simulink model "bms_vcu_inverter_can_simulink"  (R2025b)
settings: Solver=VariableStepAuto  StartTime=0.0  StopTime=6000  RelTol=1e-3
undefined symbols (not defined in the file): Ireq, Qcell, R0cell, R1cell, R2cell, SOC0, tau1, tau2
libraries: nesl_utility x6, canmsglib x6, simulink x4, fl_lib x4, batteryecm_lib x1
settings Model: Creator=User  LastModifiedBy=User

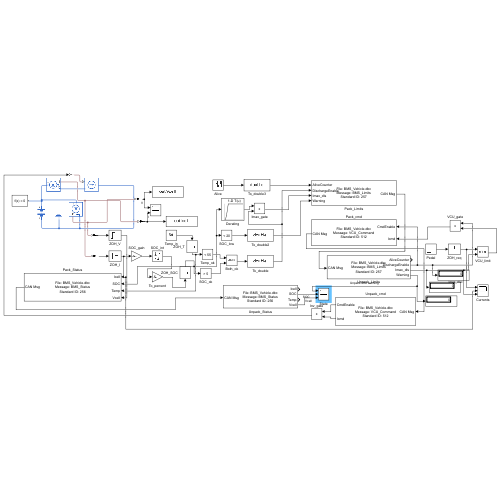
[thumbnail: Simulink's stored preview of the top-level diagram]
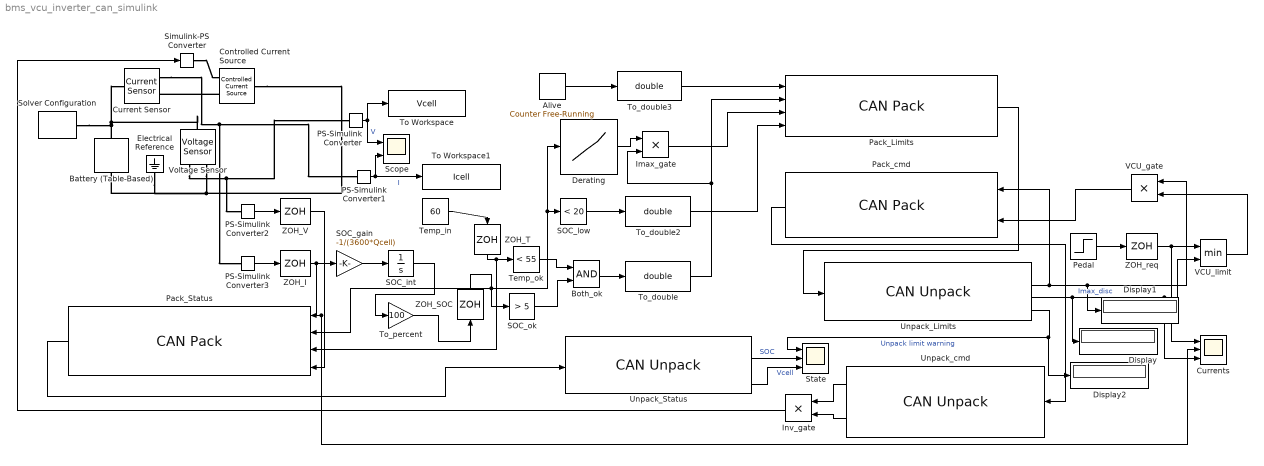
== system bms_vcu_inverter_can_simulink ==
  Alive : simulink/Sources/Counter Free-Running  NumBits=8  tsamp=0.1
  Battery (Table-Based) : batteryecm_lib/Battery (Table-Based)  SOC_vec=[0 0.2 0.5 0.8 1.0]  T_dependence=simscape.enum.tablebattery.temperature_dependence.no  prm_dir=simscape.enum.tablebattery.prm_dir.noCurrentDirectionality  T_vec=[278, 293, 313] K  V0_mat=[3.49, 3.5, 3.51; 3.55, 3.57, 3.56; 3.62, 3.63, 3.64; 3.71, 3.71, 3.72; 3.91, 3.93, 3.94; 4.07, 4.08, 4.08; 4.19, 4.19, 4.19] V  V0_vec=[3.0 3.5 3.7 4.0 4.2] V  V_range=[0, inf] V  R0_mat=[.0117, .0085, .009; .011, .0085, .009; .0114, .0087, .0092; .0107, .0082, .0088; .0107, .0083, .0091; .0113, .0085, .0089; .0116, .0085, .0089] Ohm  R0_vec=R0cell*ones(1,5) Ohm  R0_dis_mat=[.0117, .0085, .009; .011, .0085, .009; .0114, .0087, .0092; .0107, .0082, .0088; .0107, .0083, .0091; .0113, .0085, .0089; .0116, .0085, .0089] Ohm  R0_dis_vec=[.0085, .0085, .0087, .0082, .0083, .0085, .0085] Ohm  R0_ch_mat=[.0117, .0085, .009; .011, .0085, .009; .0114, .0087, .0092; .0107, .0082, .0088; .0107, .0083, .0091; .0113, .0085, .0089; .0116, .0085, .0089] Ohm  R0_ch_vec=[.0085, .0085, .0087, .0082, .0083, .0085, .0085] Ohm  AH=Qcell A*hr  prm_leak=simscape.enum.tablebattery.prm_leak.disabled  Rleak_vec=[8000, 7000, 6000] Ohm  Rleak=7e3 Ohm  extrapolation_option=simscape.enum.extrapolation.nearest  SOC_port=simscape.enum.tablebattery.enable.no  prm_dyn=simscape.enum.tablebattery.prm_dyn.rc2  R1_mat=[.0109, .0029, .0013; .0069, .0024, .0012; .0047, .0026, .0013; .0034, .0016, .001; .0033, .0023, .0014; .0033, .0018, .0011; .0028, .0017, .0011] Ohm  R1_vec=R1cell*ones(1,5) Ohm  tau1_mat=[20, 36, 39; 31, 45, 39; 109, 105, 61; 36, 29, 26; 59, 77, 67; 40, 33, 29; 25, 39, 33] s  tau1_vec=tau1*ones(1,5) s  R2_mat=[.0109, .0029, .0013; .0069, .0024, .0012; .0047, .0026, .0013; .0034, .0016, .001; .0033, .0023, .0014; .0033, .0018, .0011; .0028, .0017, .0011] Ohm  R2_vec=R2cell*ones(1,5) Ohm  tau2_mat=[20, 36, 39; 31, 45, 39; 109, 105, 61; 36, 29, 26; 59, 77, 67; 40, 33, 29; 25, 39, 33] s  tau2_vec=tau2*ones(1,5) s  R3_mat=[.0109, .0029, .0013; .0069, .0024, .0012; .0047, .0026, .0013; .0034, .0016, .001; .0033, .0023, .0014; .0033, .0018, .0011; .0028, .0017, .0011] Ohm  R3_vec=[.0029, .0024, .0026, .0016, .0023, .0018, .0017] Ohm  tau3_mat=[20, 36, 39; 31, 45, 39; 109, 105, 61; 36, 29, 26; 59, 77, 67; 40, 33, 29; 25, 39, 33] s  tau3_vec=[36, 45, 105, 29, 77, 33, 39] s  R4_mat=[.0109, .0029, .0013; .0069, .0024, .0012; .0047, .0026, .0013; .0034, .0016, .001; .0033, .0023, .0014; .0033, .0018, .0011; .0028, .0017, .0011] Ohm  R4_vec=[.0029, .0024, .0026, .0016, .0023, .0018, .0017] Ohm  tau4_mat=[20, 36, 39; 31, 45, 39; 109, 105, 61; 36, 29, 26; 59, 77, 67; 40, 33, 29; 25, 39, 33] s  tau4_vec=[36, 45, 105, 29, 77, 33, 39] s  R5_mat=[.0109, .0029, .0013; .0069, .0024, .0012; .0047, .0026, .0013; .0034, .0016, .001; .0033, .0023, .0014; .0033, .0018, .0011; .0028, .0017, .0011] Ohm  R5_vec=[.0029, .0024, .0026, .0016, .0023, .0018, .0017] Ohm  tau5_mat=[20, 36, 39; 31, 45, 39; 109, 105, 61; 36, 29, 26; 59, 77, 67; 40, 33, 29; 25, 39, 33] s  tau5_vec=[36, 45, 105, 29, 77, 33, 39] s  prm_fade=simscape.enum.tablebattery.prm_fade.disabled  N0=100  dV0=0  dR0=0  dAH=0  dRleak=0  dR1=0  dR2=0  dR3=0  dR4=0  dR5=0  N0vec=[0, 100, 200, 300]  Tfadevec=[298.15, 323.15] K  dV0vec=[0, 0, 0, 0]  dR0vec=[0, 0, 0, 0]  dAHvec=[0, 0, 0, 0]  dRleakvec=[0, 0, 0, 0]  dR1vec=[0, 0, 0, 0]  dR2vec=[0, 0, 0, 0]  dR3vec=[0, 0, 0, 0]  dR4vec=[0, 0, 0, 0]  dR5vec=[0, 0, 0, 0]  dV0mat=[0, 0; 0, 0; 0, 0; 0, 0]  dR0mat=[0, 0; 0, 0; 0, 0; 0, 0]  dAHmat=[0, 0; 0, 0; 0, 0; 0, 0]  dRleakmat=[0, 0; 0, 0; 0, 0; 0, 0]  dR1mat=[0, 0; 0, 0; 0, 0; 0, 0]  dR2mat=[0, 0; 0, 0; 0, 0; 0, 0]  dR3mat=[0, 0; 0, 0; 0, 0; 0, 0]  dR4mat=[0, 0; 0, 0; 0, 0; 0, 0]  dR5mat=[0, 0; 0, 0; 0, 0; 0, 0]  prm_age_modeling=simscape.enum.tablebattery.prm_age_modeling.equation  storage_dt_age_vec=[0] d  storage_T_age_vec=[273] K  prm_age_OCV=simscape.enum.tablebattery.prm_age_OCV.OCV  OCV_age=0.9  SOC_age=0.6  prm_age_resistance=simscape.enum.tablebattery.prm_age.disabled  OCV_scaling_age_resistance=2.2134e6  OCV_offset_age_resistance=1.632e6  temp_exp_age_resistance=0.515833569 V  t_exp_age_resistance=0.75  T_age_vec_resistance=[273.15, 298.15, 323.15] K  dt_age_vec_resistance=[0, 90, 180, 270] d  dR0_age_vec=[0, 0, 0]  t_meas_dR0_age=100 d  dR0_age_mat=[0, 0, 0; 0, 0, 0; 0, 0, 0; 0, 0, 0]  prm_age_capacity=simscape.enum.tablebattery.prm_age.disabled  OCV_scaling_age_capacity=1.5097e07  OCV_offset_age_capacity=8.3625e06  temp_exp_age_capacity=0.6011 V  t_exp_age_capacity=0.75  T_age_vec_capacity=[273.15, 298.15, 323.15] K  dt_age_vec_capacity=[0, 90, 180, 270] d  dAH_age_vec=[0, 0, 0]  t_meas_dAH_age=100 d  dAH_age_mat=[0, 0, 0; 0, 0, 0; 0, 0, 0; 0, 0, 0]  thermal_port=simscape.enum.thermaleffects.omit  temperature=298.15 K  thermal_mass=100 J/K  i_specify=off  i_priority=None  i=0 A  i_nominal_specify=off  i_nominal_value=1  i_nominal_unit=A  v_specify=off  v_priority=None  v=0 V  v_nominal_specify=off  v_nominal_value=1  v_nominal_unit=V  stateOfCharge_specify=on  stateOfCharge_priority=High  stateOfCharge=SOC0  stateOfCharge_nominal_specify=off  stateOfCharge_nominal_value=1  stateOfCharge_nominal_unit=1  num_cycles_specify=off  num_cycles_priority=High  num_cycles=0  num_cycles_nominal_specify=off  num_cycles_nominal_value=1  num_cycles_nominal_unit=1  cell_temperature_specify=off  cell_temperature_priority=High  cell_temperature=298.15 K  cell_temperature_nominal_specify=off  cell_temperature_nominal_value=1  cell_temperature_nominal_unit=K
      settings: InternalSimscapePortConfiguration="{\"Bottom\":[],\"Left\":[{\"id\":\"p\",\"label\":\"+\",\"type\":\"foundation.electrical.electrical\"}],\"Right\":[{\"id\":\"n\",\"label\":\"-\",\"type\":\"foundation.electrical.electrical\"}],\"Top\":[]}"
      settings: LibrarySourceBlock=|
      | batt_lib/Cells/Battery
      | (Table-Based)
  Both_ok : Logic  AllPortsSameDT=off  OutDataTypeStr=boolean
  Controlled Current Source : fl_lib/Electrical/Electrical Sources/Controlled Current Source
  Current Sensor : fl_lib/Electrical/Electrical Sensors/Current Sensor
  Currents : Scope  NumInputPorts=3
      settings: ActiveDisplayYMinimum=-0.74999999999999978  ActiveDisplayYMaximum=6.75
  Derating : Lookup_n-D  NumberOfTableDimensions=1  BreakpointsForDimension1=[0 5 10 20 100]  Table=[0 0 1.5 6 6]  InternalRulePriority=Speed  RndMeth=Simplest
  Display : Display
  Display1 : Display
  Display2 : Display
  Electrical Reference : fl_lib/Electrical/Electrical Elements/Electrical Reference
  Imax_gate : Product
  Inv_gate : Product
  PS-Simulink Converter{,1..3} (4 alike) : nesl_utility/PS-Simulink Converter  PhysicalDomain=network_engine_domain  SubClassName=ps_output  LeftPortType=input  RightPortType=output  PseudoPeriodic=off  Frequencies=[]  VectorFormat=inherit  Unit=inherit  AffineConversion=off
  Pack_Limits : canmsglib/CAN Pack  CANdbFile=C:\Users\User\Documents\MATLAB\BMS_Vehicle.dbc  MsgList=BMS_Limits  MsgName=BMS_Limits  MsgIDType=Standard (11-bit identifier)  MsgIdentifier=257  CANIDInput=off  MsgLength=8  Remote=off  ApplyMinMax=off  BusOutput=off  SignalInfo={'AliveCounter','32','8','LE','unsigned','Standard','0','1','0','0','255';'DischargeEnable','16','8','LE','unsigned','Standard','0','1','0','0','1';'Imax_dis','0','16','LE','unsigned','Standard','0','0.1','0','0','6553.5';'Warning','24','8','LE','unsigned','Standard','0','1','0','0','3'}
      settings: LibrarySourceBlock=c2000lib/Target Communication/CAN Pack  DataFormat=CANdb specified signals
  Pack_Status : canmsglib/CAN Pack  CANdbFile=C:\Users\User\Documents\MATLAB\BMS_Vehicle.dbc  MsgList=BMS_Status  MsgName=BMS_Status  MsgIDType=Standard (11-bit identifier)  MsgIdentifier=256  CANIDInput=off  MsgLength=8  Remote=off  ApplyMinMax=off  BusOutput=off  SignalInfo={'Icell','16','16','LE','signed','Standard','0','0.1','0','-3276.8','3276.7';'SOC','32','8','LE','unsigned','Standard','0','0.5','0','0','127.5';'Temp','40','8','LE','unsigned','Standard','0','1','-40','-40','215';'Vcell','0','16','LE','unsigned','Standard','0','0.001','0','0','65.535'}
      settings: LibrarySourceBlock=c2000lib/Target Communication/CAN Pack  DataFormat=CANdb specified signals
  Pack_cmd : canmsglib/CAN Pack  CANdbFile=C:\Users\User\Documents\MATLAB\BMS_Vehicle.dbc  MsgList=VCU_Command  MsgName=VCU_Command  MsgIDType=Standard (11-bit identifier)  MsgIdentifier=512  CANIDInput=off  MsgLength=8  Remote=off  ApplyMinMax=off  BusOutput=off  SignalInfo={'CmdEnable','16','8','LE','unsigned','Standard','0','1','0','0','1';'Icmd','0','16','LE','unsigned','Standard','0','0.1','0','0','6553.5'}
      settings: LibrarySourceBlock=c2000lib/Target Communication/CAN Pack  DataFormat=CANdb specified signals
  Pedal : Step  Time=10  After=Ireq  SampleTime=0
  SOC_gain : Gain  Gain=-1/(3600*Qcell)
  SOC_int : Integrator  InitialCondition=SOC0  LimitOutput=on  UpperSaturationLimit=1  LowerSaturationLimit=0
  SOC_low : simulink/Logic and Bit Operations/Compare To Constant  relop=<  const=20  OutDataTypeStr=boolean
  SOC_ok : simulink/Logic and Bit Operations/Compare To Constant  relop=>  const=5  OutDataTypeStr=boolean
  Scope : Scope  NumInputPorts=2
      settings: ActiveDisplayYMinimum=3.598991707315359  ActiveDisplayYMaximum=4.2008919512210277
  Simulink-PS Converter : nesl_utility/Simulink-PS Converter  PhysicalDomain=network_engine_domain  SubClassName=ps_input  LeftPortType=input  RightPortType=output  PseudoPeriodic=off  Frequencies=[]  NoiseDistribution=none  NoiseParameters=[]  Unit=1  AffineConversion=off  FilteringAndDerivatives=provide  SimscapeFilterOrder=1  InputFilterTimeConstant=0.001  UdotUserProvided=0
  Solver Configuration : nesl_utility/Solver Configuration  PhysicalDomain=network_engine_domain  SubClassName=solver  LeftPortType=input  RightPortType=generic  Tones=[]  Harmonics=[]  SimulateNoise=off  Profile=off  UseLocalSampling=off  EnableSwitchedLinearOptims=on  FrequencyDomain=off  UseCCode=off  RelTol=0.001  AbsTol=0.001  MinStep=1e-09  ToWorkspace=off  RevertToSquareIcSolve=off  NumHomotopyIterations=100  PhasorMode=off  PhasorModeNumHarmonics=1  ConsistencySolver=NEWTON_XTOL_AFTER_FTOL  IndexReductionMethod=DerivativeReplacement  DoDC=off  ResidualTolerance=1e-09  ConsistencyTolSource=GLOBAL  ConsistencyAbsTol=0.001  ConsistencyRelTol=0.001  ConsistencyTolFactor=0.001  UseLocalSolver=off  LocalSolverChoice=NE_BACKWARD_EULER_ADVANCER  ResolveIndetEquations=on  FunctionEvalNumThread=1  LocalSolverSampleTime=0.001  DoFixedCost=off  MaxNonlinIter=3  MaxModeIter=2  ComputeImpulses=off  ImpulseIterations=2  LinearAlgebra=auto  LinearAlgebraNumThread=0  EquationFormulation=NE_TIME_EF  DelaysMemoryBudget=1024  AutomaticFiltering=on  FilteringTimeConstant=0.001  PartitionStorageMethod=AS_NEEDED  PartitionMemoryBudget=1024  PartitionMethod=ROBUST  MultibodyUseLocalSolver=off  MultibodyLocalSolverChoice=ODE1  MultibodyLocalSolverSampleTime=0.001
  State : Scope  NumInputPorts=3
      settings: ActiveDisplayYMinimum=-1  ActiveDisplayYMaximum=1  DataLoggingVariableName=ScopeData2
  Temp_in : Constant  Value=60
  Temp_ok : simulink/Logic and Bit Operations/Compare To Constant  relop=<  const=55  OutDataTypeStr=boolean
  To Workspace : ToWorkspace  VariableName=Vcell  SaveFormat=Timeseries  SampleTime=-1
  To Workspace1 : ToWorkspace  VariableName=Icell  SaveFormat=Timeseries  SampleTime=-1
  To_double : DataTypeConversion  OutDataTypeStr=double  SaturateOnIntegerOverflow=off  RndMeth=Floor
  To_double2 : DataTypeConversion  OutDataTypeStr=double  SaturateOnIntegerOverflow=off  RndMeth=Floor
  To_double3 : DataTypeConversion  OutDataTypeStr=double  SaturateOnIntegerOverflow=off  RndMeth=Floor
  To_percent : Gain  Gain=100
  Unpack_Limits : canmsglib/CAN Unpack  CANdbFile=C:\Users\User\Documents\MATLAB\BMS_Vehicle.dbc  MsgList=BMS_Limits  MsgName=BMS_Limits  MsgIDType=Standard (11-bit identifier)  MsgIdentifier=257  MsgLength=8  SignalInfo={'AliveCounter','32','8','LE','unsigned','Standard','0','1','0','0','255';'DischargeEnable','16','8','LE','unsigned','Standard','0','1','0','0','1';'Imax_dis','0','16','LE','unsigned','Standard','0','0.1','0','0','6553.5';'Warning','24','8','LE','unsigned','Standard','0','1','0','0','3'}  IDPort=off  TimestampPort=off  ErrorPort=off  RemotePort=off  LengthPort=off  StatusPort=off  ApplyMinMax=off
      settings: LibrarySourceBlock=canlib/CAN Unpack  DataFormat=CANdb specified signals
  Unpack_Status : canmsglib/CAN Unpack  CANdbFile=C:\Users\User\Documents\MATLAB\BMS_Vehicle.dbc  MsgList=BMS_Status  MsgName=BMS_Status  MsgIDType=Standard (11-bit identifier)  MsgIdentifier=256  MsgLength=8  SignalInfo={'Icell','16','16','LE','signed','Standard','0','0.1','0','-3276.8','3276.7';'SOC','32','8','LE','unsigned','Standard','0','0.5','0','0','127.5';'Temp','40','8','LE','unsigned','Standard','0','1','-40','-40','215';'Vcell','0','16','LE','unsigned','Standard','0','0.001','0','0','65.535'}  IDPort=off  TimestampPort=off  ErrorPort=off  RemotePort=off  LengthPort=off  StatusPort=off  ApplyMinMax=off
      settings: LibrarySourceBlock=canlib/CAN Unpack  DataFormat=CANdb specified signals
  Unpack_cmd : canmsglib/CAN Unpack  CANdbFile=C:\Users\User\Documents\MATLAB\BMS_Vehicle.dbc  MsgList=VCU_Command  MsgName=VCU_Command  MsgIDType=Standard (11-bit identifier)  MsgIdentifier=512  MsgLength=8  SignalInfo={'CmdEnable','16','8','LE','unsigned','Standard','0','1','0','0','1';'Icmd','0','16','LE','unsigned','Standard','0','0.1','0','0','6553.5'}  IDPort=off  TimestampPort=off  ErrorPort=off  RemotePort=off  LengthPort=off  StatusPort=off  ApplyMinMax=off
      settings: LibrarySourceBlock=canlib/CAN Unpack  DataFormat=CANdb specified signals
  VCU_gate : Product
  VCU_limit : MinMax  Inputs=2
  Voltage Sensor : fl_lib/Electrical/Electrical Sensors/Voltage Sensor
  ZOH_I : ZeroOrderHold  SampleTime=0.1
  ZOH_SOC : ZeroOrderHold  SampleTime=0.1
  ZOH_T : ZeroOrderHold  SampleTime=0.1
  ZOH_V : ZeroOrderHold  SampleTime=0.1
  ZOH_req : ZeroOrderHold  SampleTime=0.1
  wires:
  PS-Simulink Converter/1 -> Scope/1, To Workspace/1  "V"
  PS-Simulink Converter1/1 -> Scope/2, To Workspace1/1  "I"
  PS-Simulink Converter2/1 -> ZOH_V/1
  PS-Simulink Converter3/1 -> ZOH_I/1
  ZOH_I/1 -> Currents/2, Pack_Status/1, SOC_gain/1
  SOC_gain/1 -> SOC_int/1
  SOC_int/1 -> To_percent/1
  To_percent/1 -> ZOH_SOC/1
  Temp_in/1 -> ZOH_T/1
  ZOH_SOC/1 -> Pack_Status/2, Derating/1, SOC_low/1, SOC_ok/1
  ZOH_T/1 -> Pack_Status/3, Temp_ok/1
  SOC_ok/1 -> Both_ok/2
  Temp_ok/1 -> Both_ok/1
  Both_ok/1 -> To_double/1
  SOC_low/1 -> To_double2/1
  Derating/1 -> Imax_gate/1
  To_double/1 -> Pack_Limits/2, Imax_gate/2
  Alive/1 -> To_double3/1
  ZOH_V/1 -> Pack_Status/4
  Imax_gate/1 -> Pack_Limits/3
  To_double2/1 -> Pack_Limits/4
  To_double3/1 -> Pack_Limits/1
  Pack_Status/1 -> Unpack_Status/1
  Pack_Limits/1 -> Unpack_Limits/1
  Pedal/1 -> ZOH_req/1
  ZOH_req/1 -> Currents/1, VCU_limit/1
  Unpack_Limits/3 -> Display/1, Currents/3, VCU_limit/2  "Imax_disc"
  VCU_limit/1 -> VCU_gate/2
  Unpack_Limits/2 -> Pack_cmd/1, Display1/1, VCU_gate/1
  VCU_gate/1 -> Pack_cmd/2
  Pack_cmd/1 -> Unpack_cmd/1
  Unpack_cmd/1 -> Inv_gate/1
  Unpack_cmd/2 -> Inv_gate/2
  Inv_gate/1 -> Simulink-PS Converter/1
  Unpack_Status/2 -> State/2  "SOC"
  Unpack_Status/4 -> State/3  "Vcell"
  Unpack_Limits/4 -> Display2/1, State/1  "Unpack limit warning"
  connections:
  Battery (Table-Based)/LConn1 -- Voltage Sensor/LConn1 -- Current Sensor/LConn1 -- Solver Configuration/RConn1
  Controlled Current Source/LConn1 -- Electrical Reference/LConn1 -- Battery (Table-Based)/RConn1 -- Voltage Sensor/RConn2
  Controlled Current Source/RConn2 -- Current Sensor/RConn2
  Simulink-PS Converter/RConn1 -- Controlled Current Source/RConn1
  Voltage Sensor/RConn1 -- PS-Simulink Converter2/LConn1 -- PS-Simulink Converter/LConn1
  Current Sensor/RConn1 -- PS-Simulink Converter3/LConn1 -- PS-Simulink Converter1/LConn1
